simulink model "bms"  (R2025b)
settings: configuration reference "cfgBMS" (kept outside this file)
values from neighbouring files (symbols this model uses):
  BMS_iPlausMax = 200.0    [bms.sldd]
  BMS_iRest = 0.2    [bms.sldd]
  BMS_nRetryMax = 3.0    [bms.sldd]
  BMS_ocvSoc : value not decoded    [bms.sldd]
  BMS_ocvV : value not decoded    [bms.sldd]
  BMS_Qnom = 23.45    [bms.sldd]
  BMS_soaLim : value not decoded    [bms.sldd]
  BMS_socMismatchTol = 0.1    [bms.sldd]
  BMS_tCloseMax = 0.5    [bms.sldd]
  BMS_tDiagClear = 1.0    [bms.sldd]
  BMS_tDiagSet = 0.5    [bms.sldd]
  BMS_tInitMax = 10.0    [bms.sldd]
  BMS_tInitSettle = 1.0    [bms.sldd]
  BMS_tPlausRange : value not decoded    [bms.sldd]
  BMS_tPowerPress = 1.0    [bms.sldd]
  BMS_tRecover = 5.0    [bms.sldd]
  BMS_tRelax = 7200.0    [bms.sldd]
  BMS_tResetPress = 3.0    [bms.sldd]
  BMS_tRestRecal = 600.0    [bms.sldd]
  BMS_tRetryReset = 60.0    [bms.sldd]
  BMS_Ts = 0.1    [bms.sldd]
  BMS_tStale : value not decoded    [bms.sldd]
  BMS_vPlausRange : value not decoded    [bms.sldd]
libraries: simulink x4
(part 2 of 2)

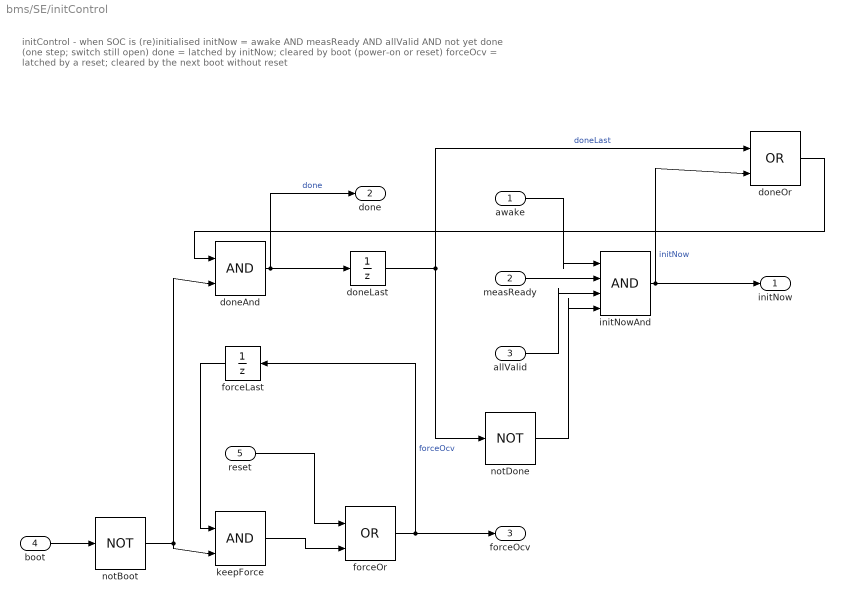
== system bms/SE/initControl ==
  note: initControl - when SOC is (re)initialised
      |   initNow  = awake AND measReady AND allValid AND not yet done   (one step; switch still open)
      |   done     = latched by initNow; cleared by boot (power-on or reset)
      |   forceOcv = latched by a reset; cleared by the next boot without reset
  awake : Inport
  measReady : Inport  Port=2
  allValid : Inport  Port=3
  boot : Inport  Port=4
  reset : Inport  Port=5
  doneAnd : Logic  IconShape=distinctive
  doneLast : UnitDelay  InitialCondition=false  SampleTime=-1
  doneOr : Logic  Operator=OR  IconShape=distinctive
  forceLast : UnitDelay  InitialCondition=false  SampleTime=-1
  forceOr : Logic  Operator=OR  IconShape=distinctive
  initNowAnd : Logic  Inputs=4  IconShape=distinctive
  keepForce : Logic  IconShape=distinctive
  notBoot : Logic  Operator=NOT  IconShape=distinctive
  notDone : Logic  Operator=NOT  IconShape=distinctive
  initNow : Outport
  done : Outport  Port=2
  forceOcv : Outport  Port=3
  wires:
  forceOr/1 -> forceLast/1, forceOcv/1  "forceOcv"
  keepForce/1 -> forceOr/2
  reset/1 -> forceOr/1
  forceLast/1 -> keepForce/1
  doneAnd/1 -> doneLast/1, done/1  "done"
  notBoot/1 -> keepForce/2, doneAnd/2
  doneOr/1 -> doneAnd/1
  boot/1 -> notBoot/1
  initNowAnd/1 -> doneOr/2, initNow/1  "initNow"
  notDone/1 -> initNowAnd/4
  allValid/1 -> initNowAnd/3
  measReady/1 -> initNowAnd/2
  awake/1 -> initNowAnd/1
  doneLast/1 -> doneOr/1, notDone/1  "doneLast"

== system bms/SE/ocvToSoc ==
  note: ocvToSoc - SOC from each group's open-circuit voltage
      |   In vGroup 13x1 V | Out socOcv 13x1 (0..1) | Table BMS_ocvV -> BMS_ocvSoc, linear, clipped at the ends
  vGroup : Inport
  ocvTable : Lookup_n-D  NumberOfTableDimensions=1  BreakpointsForDimension1=BMS_ocvV  Table=BMS_ocvSoc  ExtrapMethod=Clip  InternalRulePriority=Speed  RndMeth=Simplest
  socOcv : Outport
  wires:
  ocvTable/1 -> socOcv/1  "socOcv"
  vGroup/1 -> ocvTable/1  "vGroup"

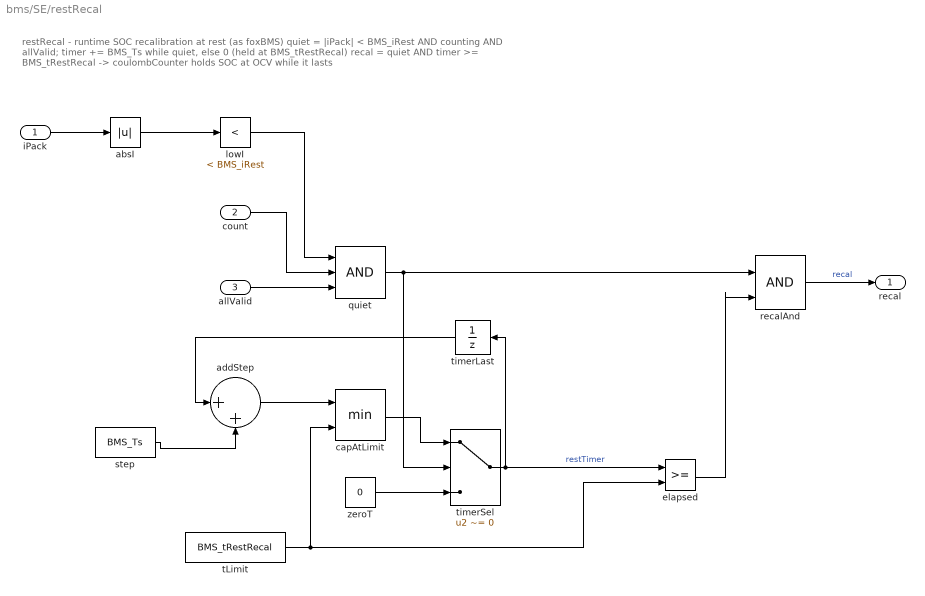
== system bms/SE/restRecal ==
  note: restRecal - runtime SOC recalibration at rest (as foxBMS)
      |   quiet = |iPack| < BMS_iRest AND counting AND allValid;  timer += BMS_Ts while quiet, else 0 (held at BMS_tRestRecal)
      |   recal = quiet AND timer >= BMS_tRestRecal  ->  coulombCounter holds SOC at OCV while it lasts
  iPack : Inport
  count : Inport  Port=2
  allValid : Inport  Port=3
  absI : Abs
  addStep : Sum  Inputs=|++
  capAtLimit : MinMax  Inputs=2
  elapsed : RelationalOperator
  lowI : simulink/Logic and Bit Operations/Compare To Constant  relop=<  const=BMS_iRest  OutDataTypeStr=boolean
  quiet : Logic  Inputs=3  IconShape=distinctive
  recalAnd : Logic  IconShape=distinctive
  step : Constant  Value=BMS_Ts
  tLimit : Constant  Value=BMS_tRestRecal
  timerLast : UnitDelay  SampleTime=-1
  timerSel : Switch  Criteria=u2 ~= 0
  zeroT : Constant  Value=0
  recal : Outport
  wires:
  recalAnd/1 -> recal/1  "recal"
  elapsed/1 -> recalAnd/2
  timerSel/1 -> elapsed/1, timerLast/1  "restTimer"
  zeroT/1 -> timerSel/3
  quiet/1 -> recalAnd/1, timerSel/2
  capAtLimit/1 -> timerSel/1
  tLimit/1 -> elapsed/2, capAtLimit/2
  addStep/1 -> capAtLimit/1
  step/1 -> addStep/2
  timerLast/1 -> addStep/1
  allValid/1 -> quiet/3
  count/1 -> quiet/2
  lowI/1 -> quiet/1
  absI/1 -> lowI/1
  iPack/1 -> absI/1

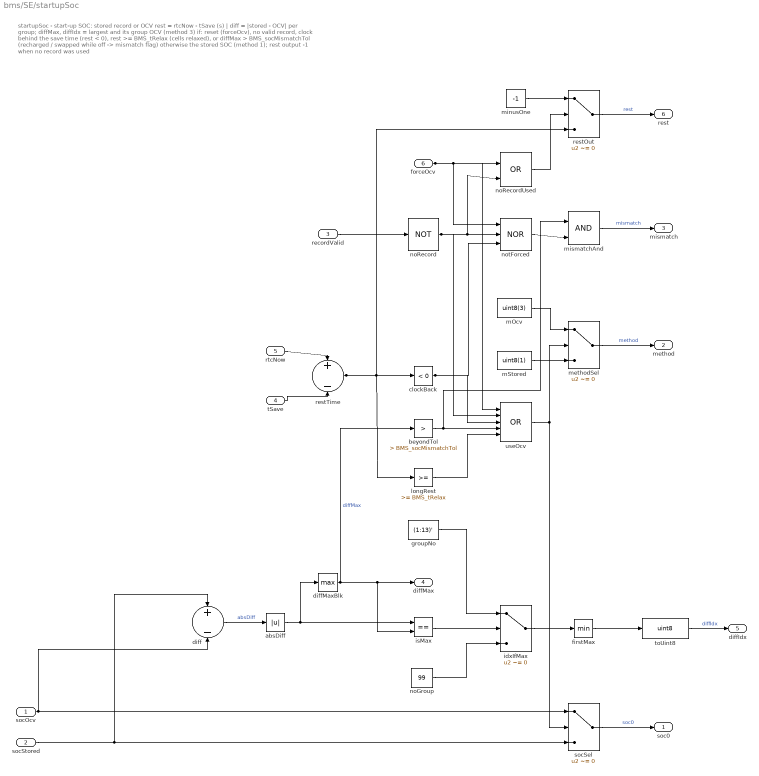
== system bms/SE/startupSoc ==
  note: startupSoc - start-up SOC: stored record or OCV
      |   rest = rtcNow - tSave (s) | diff = |stored - OCV| per group; diffMax, diffIdx = largest and its group
      |   OCV (method 3) if: reset (forceOcv), no valid record, clock behind the save time (rest < 0),
      |      rest >= BMS_tRelax (cells relaxed), or diffMax > BMS_socMismatchTol (recharged / swapped while off -> mismatch flag)
      |   otherwise the stored SOC (method 1);  rest output -1 when no record was used
  socOcv : Inport
  socStored : Inport  Port=2
  recordValid : Inport  Port=3
  tSave : Inport  Port=4
  rtcNow : Inport  Port=5
  forceOcv : Inport  Port=6
  absDiff : Abs
  beyondTol : simulink/Logic and Bit Operations/Compare To Constant  relop=>  const=BMS_socMismatchTol  OutDataTypeStr=boolean
  clockBack : simulink/Logic and Bit Operations/Compare To Constant  relop=<  const=0  OutDataTypeStr=boolean
  diff : Sum  Inputs=+-
  diffMaxBlk : MinMax  Function=max
  firstMax : MinMax
  groupNo : Constant  Value=(1:13)'
  idxIfMax : Switch  Criteria=u2 ~= 0
  isMax : RelationalOperator  Operator===
  longRest : simulink/Logic and Bit Operations/Compare To Constant  relop=>=  const=BMS_tRelax  OutDataTypeStr=boolean
  mOcv : Constant  Value=uint8(3)
  mStored : Constant  Value=uint8(1)
  methodSel : Switch  Criteria=u2 ~= 0
  minusOne : Constant  Value=-1
  mismatchAnd : Logic  IconShape=distinctive
  noGroup : Constant  Value=99
  noRecord : Logic  Operator=NOT  IconShape=distinctive
  noRecordUsed : Logic  Operator=OR  IconShape=distinctive
  notForced : Logic  Operator=NOR  Inputs=3  IconShape=distinctive
  restOut : Switch  Criteria=u2 ~= 0
  restTime : Sum  Inputs=+-
  socSel : Switch  Criteria=u2 ~= 0
  toUint8 : DataTypeConversion  OutDataTypeStr=uint8
  useOcv : Logic  Operator=OR  Inputs=5  IconShape=distinctive
  soc0 : Outport
  method : Outport  Port=2
  mismatch : Outport  Port=3
  diffMax : Outport  Port=4
  diffIdx : Outport  Port=5
  rest : Outport  Port=6
  wires:
  methodSel/1 -> method/1  "method"
  mStored/1 -> methodSel/3
  mOcv/1 -> methodSel/1
  socSel/1 -> soc0/1  "soc0"
  useOcv/1 -> methodSel/2, socSel/2
  longRest/1 -> useOcv/5
  rtcNow/1 -> restTime/1
  tSave/1 -> restTime/2
  socStored/1 -> socSel/3, diff/1
  socOcv/1 -> socSel/1, diff/2
  diff/1 -> absDiff/1  "absDiff"
  absDiff/1 -> isMax/1, diffMaxBlk/1
  diffMaxBlk/1 -> beyondTol/1, diffMax/1, isMax/2  "diffMax"
  groupNo/1 -> idxIfMax/1
  isMax/1 -> idxIfMax/2
  noGroup/1 -> idxIfMax/3
  idxIfMax/1 -> firstMax/1
  firstMax/1 -> toUint8/1
  toUint8/1 -> diffIdx/1  "diffIdx"
  restTime/1 -> clockBack/1, longRest/1, restOut/3
  recordValid/1 -> noRecord/1
  forceOcv/1 -> noRecordUsed/1, useOcv/1, notForced/1
  noRecord/1 -> useOcv/2, notForced/2, noRecordUsed/2
  clockBack/1 -> notForced/3, useOcv/3
  beyondTol/1 -> useOcv/4, mismatchAnd/1
  notForced/1 -> mismatchAnd/2
  mismatchAnd/1 -> mismatch/1  "mismatch"
  minusOne/1 -> restOut/1
  noRecordUsed/1 -> restOut/2
  restOut/1 -> rest/1  "rest"

== matlab function bms/DIAG/diagFcn ==
  data: s input Bus: BMS_soaData; d output Bus: DIAG_bus; v input Bus: BMS_validData; pw input Bus: BMS_pwrData; BMS_tDiagSet parameter; BMS_tDiagClear parameter; BMS_Ts parameter
function d = diagFcn(s, v, pw, BMS_tDiagSet, BMS_tDiagClear, BMS_Ts)
% DIAG layer: debounced fault flags; nothing evaluated while off or before measReady. Logic in diagDebounce.m.
d = diagDebounce(s, v.allValid, v.measReady, BMS_tDiagSet, BMS_tDiagClear, BMS_Ts, pw.awake, pw.boot);

== matlab function bms/BMSVL/bmsvlFcn ==
  data: p input Bus: BMS_plausData; pw input Bus: BMS_pwrData; v output Bus: BMS_validData; BMS_soaLim parameter
function v = bmsvlFcn(p, pw, BMS_soaLim)
% BMSVL layer: validated values; extremes over VALID channels only. Logic in validExtremes.m.
v = validExtremes(p, BMS_soaLim, pw.boot);

== matlab function bms/LOG/logFcn ==
  data: v input Bus: BMS_validData; events output Bus: BMS_event size=6; d input Bus: DIAG_bus; p input Bus: BMS_plausData; state input Enum: BMS_state; cmd input boolean; cause input Enum: BMS_eventCode; latched input boolean; se input Bus: BMS_seData; pw input Bus: BMS_pwrData; eventCount output uint32; eventDropped output uint32; BMS_soaLim parameter; BMS_iRest parameter; BMS_socMismatchTol parameter; BMS_Ts parameter
function [events, eventCount, eventDropped] = logFcn(v, d, p, state, cmd, cause, latched, se, pw, BMS_soaLim, BMS_iRest, BMS_socMismatchTol, BMS_Ts)
% LOG layer: time-stamped INFO/MINOR/MAJOR/FAULT records. Logic in logEvents.m.
[events, eventCount, eventDropped] = logEvents(v, d, p, se, pw, state, cmd, cause, latched, BMS_soaLim, BMS_iRest, BMS_socMismatchTol, BMS_Ts);

== matlab function bms/PWR/pwrFcn ==
  data: hw input Bus: BMS_hwIn; pw output Bus: BMS_pwrData; BMS_tPowerPress parameter; BMS_tResetPress parameter; BMS_Ts parameter
function pw = pwrFcn(hw, BMS_tPowerPress, BMS_tResetPress, BMS_Ts)
% PWR layer: power and reset buttons (long presses). Logic in pwrManager.m.
pw = pwrManager(hw, BMS_tPowerPress, BMS_tResetPress, BMS_Ts);

== matlab function bms/SOA/soaFcn ==
  data: v input Bus: BMS_validData; s output Bus: BMS_soaData; BMS_soaLim parameter; BMS_iRest parameter
function s = soaFcn(v, BMS_soaLim, BMS_iRest)
% SOA layer: safe-operating-area limit checks [MOL RSL MSL]. Logic in soaCheck.m.
s = soaCheck(v, BMS_soaLim, BMS_iRest);

== matlab function bms/PLAUS/plausFcn ==
  data: m input Bus: BMS_measData; pw input Bus: BMS_pwrData; p output Bus: BMS_plausData; BMS_vPlausRange parameter; BMS_iPlausMax parameter; BMS_tPlausRange parameter; BMS_tStale parameter; BMS_Ts parameter
function p = plausFcn(m, pw, BMS_vPlausRange, BMS_iPlausMax, BMS_tPlausRange, BMS_tStale, BMS_Ts)
% PLAUS layer: per-channel plausibility (range and staleness); restarts on power-up/reset. Logic in plausCheck.m.
p = plausCheck(m, BMS_vPlausRange, BMS_iPlausMax, BMS_tPlausRange, BMS_tStale, BMS_Ts, pw.boot);

== stateflow chart bms/BMS/stateMachine ==
  state OFF
    en: state = BMS_state.OFF;
    contactorCmd = false;
  state ON
    en: retries = uint8(0);
    latched = false;
    errorCause = BMS_eventCode.NONE;
    state INITIALIZATION
      en: state = BMS_state.INITIALIZATION;
      state CHECK
        en: contactorCmd = false;
      state CLOSE
        en: contactorCmd = true;
      (default) -> CHECK
      CHECK -> CLOSE : [duration(allValid && ~anyFatal && ~contactorFb, sec) >= BMS_tInitSettle]
    state NORMAL
      en: state = BMS_state.NORMAL;
      contactorCmd = true;
      on after(BMS_tRetryReset, sec): retries = uint8(0);
    state ERROR
      en: state = BMS_state.ERROR;
      contactorCmd = false;
      retries = retries + 1;
      latched = retries >= BMS_nRetryMax;
    ON -> ON [order 1] : [boot]{retries = uint8(0); latched = false; errorCause = BMS_eventCode.NONE;}
    (default) -> INITIALIZATION
    CLOSE -> ERROR [order 2] : [after(BMS_tCloseMax, sec)]{errorCause = BMS_eventCode.SWITCH_STUCK_OPEN;}
    CLOSE -> NORMAL [order 1] : [contactorFb]
    INITIALIZATION -> ERROR [order 2] : [after(BMS_tInitMax, sec) && contactorFb]{errorCause = BMS_eventCode.SWITCH_WELDED;}
    INITIALIZATION -> ERROR [order 1] : [after(BMS_tInitMax, sec) && ~contactorFb]{errorCause = BMS_eventCode.INIT_TIMEOUT;}
    ERROR -> INITIALIZATION : [retries < BMS_nRetryMax && duration(~anyFatal, sec) >= BMS_tRecover]{errorCause = BMS_eventCode.NONE;}
    NORMAL -> ERROR [order 1] : [anyFatal]{errorCause = BMS_eventCode.DIAG_FAULT;}
    NORMAL -> ERROR [order 2] : [~contactorFb]{errorCause = BMS_eventCode.SWITCH_OPENED_UNEXPECTEDLY;}
  OFF -> ON : [awake]
  (default) -> OFF
  ON -> OFF [order 1] : [~awake]
  data: allValid input boolean; anyFatal input boolean; contactorFb input boolean; state output Enum: BMS_state =BMS_state.OFF; contactorCmd output boolean =false; retries local uint8 =0; BMS_tInitSettle parameter; BMS_tInitMax parameter; BMS_tCloseMax parameter; BMS_tRecover parameter; BMS_nRetryMax parameter; BMS_tRetryReset parameter; errorCause output Enum: BMS_eventCode =BMS_eventCode.NONE; latched output boolean =false; awake input boolean; boot input boolean
